simulink model "str_form_iii"  (R2024b)
settings: Solver=FixedStepAuto  StartTime=0.0  StopTime=max_time  FixedStep=Ts  MaxStep=0.02  RelTol=1e-3
undefined symbols (not defined in the file): coa, dVel, goc, K, max_pos, obstacles, offsets, params, pg_period, t_change1, t_change2, Ts, use_col, use_obs, wn_smpl_time
libraries: lib_vehicle_dyn x7
settings Model: Creator=simon  LastModifiedBy=simon
settings RTWCC: GPUComputeCapability=3.5

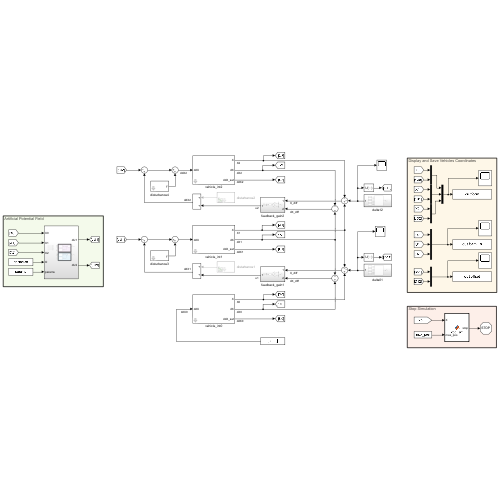
[thumbnail: Simulink's stored preview of the top-level diagram]
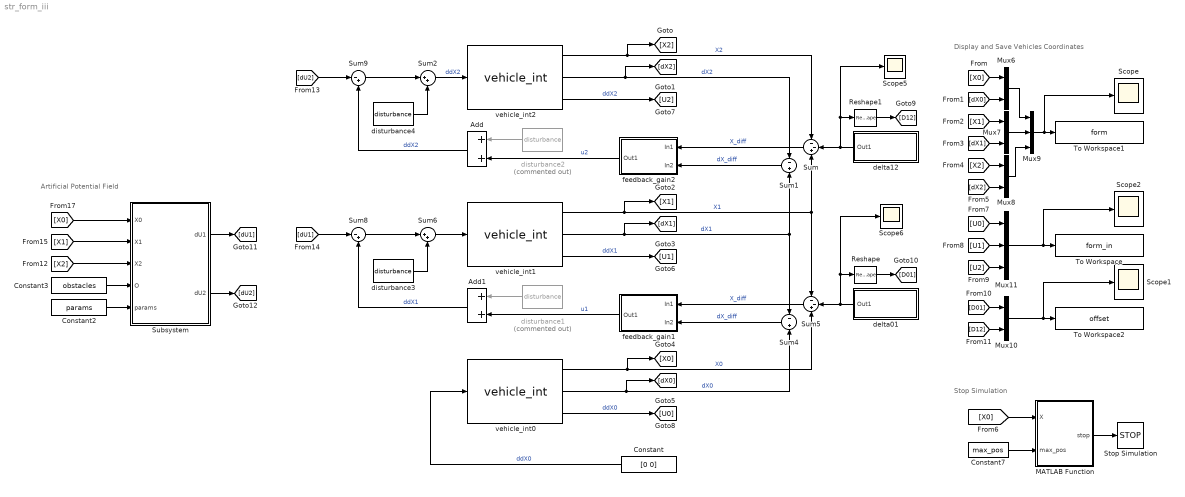
== system str_form_iii ==
  note: Artificial Potential Field
  note: Stop Simulation
  note: Display and Save Vehicles Coordinates
  Add : Sum
  Add1 : Sum
  Constant : Constant  Value=[0 0]
  Constant2 : Constant  Value=params
  Constant3 : Constant  Value=obstacles
  Constant7 : Constant  Value=max_pos
  MATLAB Function : MATLAB Function  TreatAsAtomicUnit=on
  Mux{6..8,10} (4 alike) : Mux  Inputs=2
  Mux11 : Mux  Inputs=3
  Mux9 : Mux  Inputs=3
  Reshape : Reshape
  Reshape1 : Reshape
  Scope{,1..2,5..6} (5 alike) : Scope
  Stop Simulation : Stop
  Subsystem : Subsystem
  Sum : Sum  Inputs=--+
  Sum1 : Sum  Inputs=-+
  Sum2 : Sum  Inputs=|++
  Sum4 : Sum  Inputs=-+
  Sum5 : Sum  Inputs=--+
  Sum6 : Sum  Inputs=|++
  Sum8 : Sum  Inputs=|-+
  Sum9 : Sum  Inputs=|-+
  To Workspace : ToWorkspace  VariableName=form_in  SaveFormat=Structure  SampleTime=Ts
  To Workspace1 : ToWorkspace  VariableName=form  SaveFormat=Structure  SampleTime=Ts
  To Workspace2 : ToWorkspace  VariableName=offset  SaveFormat=Structure  SampleTime=Ts
  delta01 : Subsystem
  delta12 : Subsystem
  disturbance1 : lib_vehicle_dyn/disturbance  Commented=on  wn_amp=wn_amp  wn_smpl_time=wn_smpl_time  wn_gain=wn_gain  pg_amp=pg_amp  pg_period=pg_period  pg_pw=pg_pw  pg_gain=pg_gain
  disturbance2 : lib_vehicle_dyn/disturbance  Commented=on  wn_amp=wn_amp  wn_smpl_time=1/2*wn_smpl_time  wn_gain=wn_gain  pg_amp=pg_amp  pg_period=1/2*pg_period  pg_pw=pg_pw  pg_gain=pg_gain
  disturbance3 : lib_vehicle_dyn/disturbance  wn_amp=wn_amp  wn_smpl_time=wn_smpl_time  wn_gain=wn_gain  pg_amp=pg_amp  pg_period=pg_period  pg_pw=pg_pw  pg_gain=pg_gain
  disturbance4 : lib_vehicle_dyn/disturbance  wn_amp=wn_amp  wn_smpl_time=wn_smpl_time  wn_gain=wn_gain  pg_amp=pg_amp  pg_period=pg_period  pg_pw=pg_pw  pg_gain=pg_gain
  feedback_gain1 : Subsystem
  feedback_gain2 : Subsystem
  vehicle_int0 : lib_vehicle_dyn/vehicle_int  x0=x00  y0=y00  dx0=dx00  dy0=dy00  u_sat=u_sat
  vehicle_int1 : lib_vehicle_dyn/vehicle_int  x0=x10  y0=y10  dx0=dx10  dy0=dy10  u_sat=u_sat
  vehicle_int2 : lib_vehicle_dyn/vehicle_int  x0=x20  y0=y20  dx0=dx20  dy0=dy20  u_sat=u_sat
  wires:
  vehicle_int2/2 -> Sum1/1, [dX2]  "dX2"
  Sum5/1 -> feedback_gain1/1(In1)  "X_diff"
  vehicle_int0/2 -> Sum4/2, [dX0]  "dX0"
  vehicle_int0/1 -> Sum5/3, [X0]  "X0"
  Mux6/1 -> Mux9/1
  [dX2] -> Mux8/2
  Sum1/1 -> feedback_gain2/2(In2)  "dX_diff"
  Sum4/1 -> feedback_gain1/2(In2)  "dX_diff"
  [dX1] -> Mux7/2
  [X1] -> Mux7/1
  feedback_gain1/1(Out1) -> Add1/2  "u1"
  feedback_gain2/1(Out1) -> Add/2  "u2"
  Mux8/1 -> Mux9/3
  [X0] -> Mux6/1
  [X2] -> Mux8/1
  Sum/1 -> feedback_gain2/1(In1)  "X_diff"
  MATLAB Function/1(stop) -> Stop Simulation/1
  [dX0] -> Mux6/2
  [X0] -> MATLAB Function/1(X)
  Constant7/1 -> MATLAB Function/2(max_pos)
  delta12/1(Out1) -> Scope5/1, Reshape1/1, Sum/2
  [U2] -> Mux11/3
  [U0] -> Mux11/1
  [U1] -> Mux11/2
  Mux7/1 -> Mux9/2
  Mux9/1 -> Scope/1, To Workspace1/1
  [D01] -> Mux10/1
  [D12] -> Mux10/2
  Mux10/1 -> Scope1/1, To Workspace2/1
  Mux11/1 -> Scope2/1, To Workspace/1
  Reshape1/1 -> [D12]
  Reshape/1 -> [D01]
  Add/1 -> Sum9/2  "ddX2"
  Add1/1 -> Sum8/2  "ddX1"
  Constant/1 -> vehicle_int0/1  "ddX0"
  vehicle_int2/3 -> [U2]  "ddX2"
  vehicle_int1/3 -> [U1]  "ddX1"
  vehicle_int0/3 -> [U0]  "ddX0"
  vehicle_int1/2 -> Sum4/1, Sum1/2, [dX1]  "dX1"
  Constant2/1 -> Subsystem/5(params)
  [dU1] -> Sum8/1
  Subsystem/2(dU2) -> [dU2]
  Constant3/1 -> Subsystem/4(O)
  [X2] -> Subsystem/3(X2)
  [X0] -> Subsystem/1(X0)
  [X1] -> Subsystem/2(X1)
  Subsystem/1(dU1) -> [dU1]
  vehicle_int2/1 -> [X2], Sum/1  "X2"
  vehicle_int1/1 -> [X1], Sum/3, Sum5/1  "X1"
  Sum6/1 -> vehicle_int1/1
  delta01/1(Out1) -> Scope6/1, Reshape/1, Sum5/2
  [dU2] -> Sum9/1
  disturbance2/1 -> Add/1
  disturbance1/1 -> Add1/1
  Sum2/1 -> vehicle_int2/1  "ddX2"
  Sum9/1 -> Sum2/1
  disturbance4/1 -> Sum2/2
  disturbance3/1 -> Sum6/2
  Sum8/1 -> Sum6/1

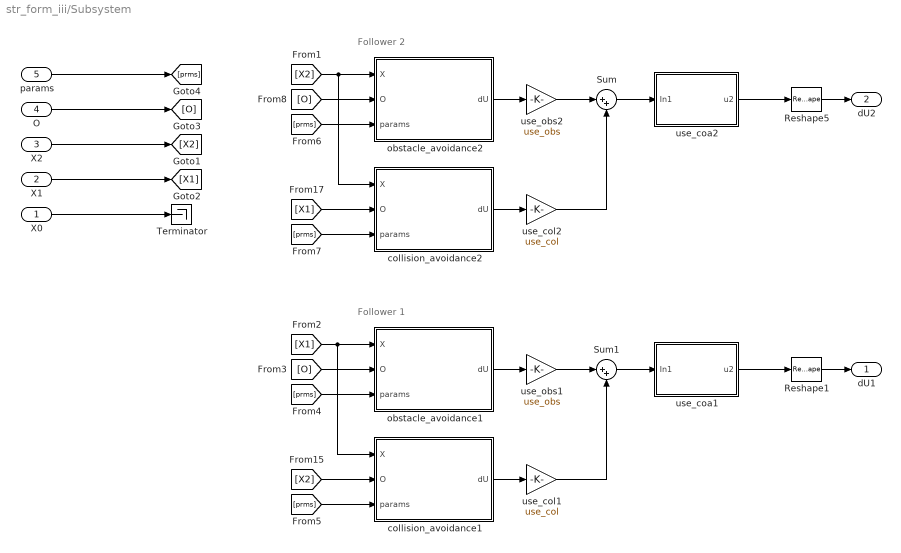
== system str_form_iii/Subsystem ==
  note: Follower 2
  note: Follower 1
  X0 : Inport
  X1 : Inport  Port=2
  X2 : Inport  Port=3
  O : Inport  Port=4
  params : Inport  Port=5
  Reshape1 : Reshape
  Reshape5 : Reshape
  Sum : Sum  Inputs=|++
  Sum1 : Sum  Inputs=|++
  Terminator : Terminator
  collision_avoidance1 : MATLAB Function  TreatAsAtomicUnit=on
  collision_avoidance2 : MATLAB Function  TreatAsAtomicUnit=on
  obstacle_avoidance1 : MATLAB Function  TreatAsAtomicUnit=on
  obstacle_avoidance2 : MATLAB Function  TreatAsAtomicUnit=on
  use_coa1 : Subsystem
  use_coa2 : Subsystem
  use_col1 : Gain  Gain=use_col
  use_col2 : Gain  Gain=use_col
  use_obs1 : Gain  Gain=use_obs
  use_obs2 : Gain  Gain=use_obs
  dU1 : Outport
  dU2 : Outport  Port=2
  wires:
  obstacle_avoidance2/1(dU) -> use_obs2/1
  Sum/1 -> use_coa2/1(In1)
  use_coa2/1(u2) -> Reshape5/1
  use_coa1/1(u2) -> Reshape1/1
  Sum1/1 -> use_coa1/1(In1)
  obstacle_avoidance1/1(dU) -> use_obs1/1
  X2/1 -> [X2]
  X1/1 -> [X1]
  params/1 -> [prms]
  collision_avoidance1/1(dU) -> use_col1/1
  collision_avoidance2/1(dU) -> use_col2/1
  X0/1 -> Terminator/1
  [X1] -> obstacle_avoidance1/1(X), collision_avoidance1/1(X)
  [prms] -> obstacle_avoidance1/3(params)
  [prms] -> collision_avoidance1/3(params)
  [prms] -> obstacle_avoidance2/3(params)
  [prms] -> collision_avoidance2/3(params)
  [O] -> obstacle_avoidance1/2(O)
  [O] -> obstacle_avoidance2/2(O)
  O/1 -> [O]
  [X2] -> collision_avoidance2/1(X), obstacle_avoidance2/1(X)
  use_obs2/1 -> Sum/1
  use_obs1/1 -> Sum1/1
  [X2] -> collision_avoidance1/2(O)
  [X1] -> collision_avoidance2/2(O)
  use_col2/1 -> Sum/2
  use_col1/1 -> Sum1/2
  Reshape5/1 -> dU2/1
  Reshape1/1 -> dU1/1

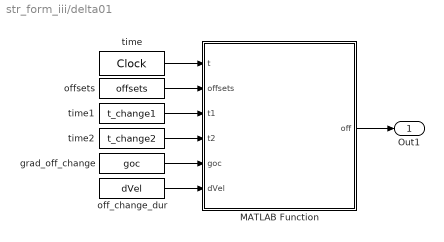
== system str_form_iii/delta01 ==
  MATLAB Function : MATLAB Function  TreatAsAtomicUnit=on
  grad_off_change : Constant  Value=goc
  off_change_dur : Constant  Value=dVel
  offsets : Constant  Value=offsets
  time : DigitalClock  SampleTime=Ts
  time1 : Constant  Value=t_change1
  time2 : Constant  Value=t_change2
  Out1 : Outport  PortDimensions=[2,1]
  wires:
  MATLAB Function/1(off) -> Out1/1
  time2/1 -> MATLAB Function/4(t2)
  offsets/1 -> MATLAB Function/2(offsets)
  time1/1 -> MATLAB Function/3(t1)
  grad_off_change/1 -> MATLAB Function/5(goc)
  time/1 -> MATLAB Function/1(t)
  off_change_dur/1 -> MATLAB Function/6(dVel)

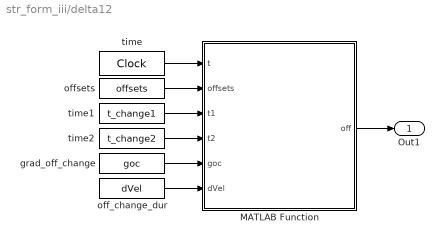
== system str_form_iii/delta12 ==
  MATLAB Function : MATLAB Function  TreatAsAtomicUnit=on
  grad_off_change : Constant  Value=goc
  off_change_dur : Constant  Value=dVel
  offsets : Constant  Value=offsets
  time : DigitalClock  SampleTime=Ts
  time1 : Constant  Value=t_change1
  time2 : Constant  Value=t_change2
  Out1 : Outport  PortDimensions=[2,1]
  wires:
  MATLAB Function/1(off) -> Out1/1
  time/1 -> MATLAB Function/1(t)
  off_change_dur/1 -> MATLAB Function/6(dVel)
  time2/1 -> MATLAB Function/4(t2)
  grad_off_change/1 -> MATLAB Function/5(goc)
  time1/1 -> MATLAB Function/3(t1)
  offsets/1 -> MATLAB Function/2(offsets)

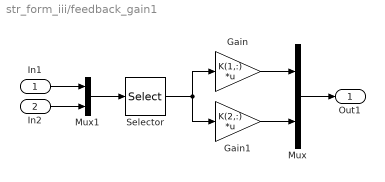
== system str_form_iii/feedback_gain1 ==
  In1 : Inport
  In2 : Inport  Port=2
  Gain : Gain  Gain=K(1,:)  Multiplication=Matrix(K*u)
  Gain1 : Gain  Gain=K(2,:)  Multiplication=Matrix(K*u)
  Mux : Mux  Inputs=2
  Mux1 : Mux  Inputs=2
  Selector : Selector  InputPortWidth=4  IndexOptions=Index vector (dialog)  Indices=[1 3 2 4]  OutputSizes=1
  Out1 : Outport
  wires:
  Mux/1 -> Out1/1
  In1/1 -> Mux1/1
  In2/1 -> Mux1/2
  Mux1/1 -> Selector/1
  Gain/1 -> Mux/1
  Gain1/1 -> Mux/2
  Selector/1 -> Gain/1, Gain1/1

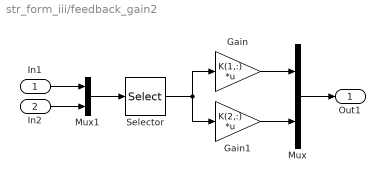
== system str_form_iii/feedback_gain2 ==
  In1 : Inport
  In2 : Inport  Port=2
  Gain : Gain  Gain=K(1,:)  Multiplication=Matrix(K*u)
  Gain1 : Gain  Gain=K(2,:)  Multiplication=Matrix(K*u)
  Mux : Mux  Inputs=2
  Mux1 : Mux  Inputs=2
  Selector : Selector  InputPortWidth=4  IndexOptions=Index vector (dialog)  Indices=[1 3 2 4]  OutputSizes=1
  Out1 : Outport
  wires:
  Mux/1 -> Out1/1
  In1/1 -> Mux1/1
  In2/1 -> Mux1/2
  Mux1/1 -> Selector/1
  Gain/1 -> Mux/1
  Gain1/1 -> Mux/2
  Selector/1 -> Gain/1, Gain1/1

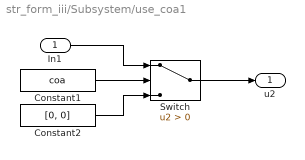
== system str_form_iii/Subsystem/use_coa1 ==
  In1 : Inport
  Constant1 : Constant  Value=coa
  Constant2 : Constant  Value=[0, 0]
  Switch : Switch  Criteria=u2 > Threshold  SaturateOnIntegerOverflow=off  InputSameDT=off
  u2 : Outport
  wires:
  In1/1 -> Switch/1
  Constant1/1 -> Switch/2
  Switch/1 -> u2/1
  Constant2/1 -> Switch/3

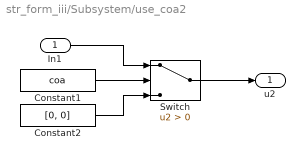
== system str_form_iii/Subsystem/use_coa2 ==
  In1 : Inport
  Constant1 : Constant  Value=coa
  Constant2 : Constant  Value=[0, 0]
  Switch : Switch  Criteria=u2 > Threshold  SaturateOnIntegerOverflow=off  InputSameDT=off
  u2 : Outport
  wires:
  In1/1 -> Switch/1
  Constant1/1 -> Switch/2
  Constant2/1 -> Switch/3
  Switch/1 -> u2/1

== matlab function str_form_iii/delta01/MATLAB Function ==
  data: t input; offsets input size=[2,6]; t1 input; t2 input; goc input; dVel input; off output
function off = variable_offset(t, offsets, t1, t2, goc, dVel)
    % get all offsets between first and second agent
    init_delta = offsets(:,1);
    l2h_delta  = offsets(:,3);
    h2l_delta  = offsets(:,5);

    goc_t1 = norm(init_delta - l2h_delta)/dVel;
    goc_t2 = norm(l2h_delta - h2l_delta)/dVel;

    % time-varying offset with smooth transition using convex combination
    if goc
        if t < t1
            off = init_delta; 
        elseif t >= t1 && t < (t1 + goc_t1)
            i = (t - t1)/goc_t1; 
            off = i.*l2h_delta + (1 - i).*init_delta;
        elseif t >= (t1 + goc_t1) && t < t2
            off = l2h_delta; 
        elseif t >= t2 && t < (t2 + goc_t2)
            i = (t - t2)/goc_t2;
            off = i.*h2l_delta + (1 - i).*l2h_delta;
        else
            off = h2l_delta;
        end
    % time-varying step offset
    else
        off = init_delta;
        if t >= t1
            off = l2h_delta;
        end
        if t >= t2
            off = h2l_delta;
        end
    end
end

== matlab function str_form_iii/MATLAB Function ==
  data: X input; stop output; max_pos input
function stop = stop_sim(X, max_pos)
    stop = 0;
    eps = 1;

    x_max = max_pos(1);
    y_max = max_pos(2);
    
    if sqrt((X(1) - x_max)^2 + (X(2) - y_max)^2) < eps
        stop = 1;
    end
end

== matlab function str_form_iii/delta12/MATLAB Function ==
  data: t input; offsets input size=[2,6]; t1 input; t2 input; goc input; dVel input; off output
function off = variable_offset(t, offsets, t1, t2, goc, dVel)
    % get all offsets between first and second agent
    delta_init = offsets(:,2);
    delta_1  = offsets(:,4);
    delta_2  = offsets(:,6);

    goc_t1 = norm(delta_init - delta_1)/dVel;
    goc_t2 = norm(delta_1 - delta_2)/dVel;

    % time-varying offset with smooth transition using convex combination
    if goc
        if t < t1
            off = delta_init; 
        elseif t >= t1 && t < (t1 + goc_t1)
            i = (t - t1)/goc_t1; 
            off = i.*delta_1 + (1 - i).*delta_init;
        elseif t >= (t1 + goc_t1) && t < t2
            off = delta_1; 
        elseif t >= t2 && t < (t2 + goc_t2)
            i = (t - t2)/goc_t2;
            off = i.*delta_2 + (1 - i).*delta_1;
        else
            off = delta_2;
        end
    % time-varying step offset
    else
        off = delta_init;
        if t >= t1
            off = delta_1;
        end
        if t >= t2
            off = delta_2;
        end
    end
end

== matlab function str_form_iii/Subsystem/collision_avoidance1 ==
  data: X input; dU output; O input; params input
function dU = col_avoid(X, O, params)
    % follower 1 -> avoid follower 2

    eta = params(1);
    rho = params(2);
    q = params(3);
    R = params(4);

    dU = zeros(2,1);

    dx = X(1) - O(1);
    dy = X(2) - O(2);
    r = hypot(dx, dy);
    r_safe = max(r, 1e-9);

    exp_arg = -((r - R)/rho)^q;
    % limit exponential function
    exp_arg = max(min(exp_arg, 60), -60);
    dU_dr = -q*eta*((r - R)^(q - 1))/(rho^q)*exp(exp_arg);

    dU(1) = dU_dr*dx/r_safe;
    dU(2) = dU_dr*dy/r_safe;
end

== matlab function str_form_iii/Subsystem/obstacle_avoidance2 ==
  data: X input; dU output; O input; params input
function dU = obs_avoid(X, O, params)

    eta = params(1);
    rho = params(2);
    q = params(3);
    
    dU = zeros(2,1);

    for i = 1:size(O,2)
        sigma = O(1:2,i);
        R = O(3,i);

        dx = X(1) - sigma(1);
        dy = X(2) - sigma(2);
        r = hypot(dx, dy);
        r_safe = max(r, 1e-9);

        exp_arg = -((r - R)/rho)^q;
        % limit exponential function
        exp_arg = max(min(exp_arg, 60), -60);
        dU_dr = -q*eta*((r - R)^(q - 1))/(rho^q)*exp(exp_arg);
    
        dU(1) = dU(1) + dU_dr*dx/r_safe;
        dU(2) = dU(2) + dU_dr*dy/r_safe;

        % s_raw = r - R;  % signed distance from the boundary
        % s = abs(s_raw); % nonnegative distance to boundary
        % sgn = 1.0; if s_raw < 0, sgn = -1.0; end
        % 
        % % dU/ds: radial derivative wrt s = |r-R|
        % dU_ds = -q*eta*s^(q-1)/rho^q*exp(-(s/rho)^q);
        % dU_dr = sgn*dU_ds;
    end
end

== matlab function str_form_iii/Subsystem/collision_avoidance2 ==
  data: X input; dU output; O input; params input
function dU = col_avoid(X, O, params)
    % follower 2 -> avoid follower 1

    eta = params(1);
    rho = params(2);
    q = params(3);
    R = params(4);

    dU = zeros(2,1);

    dx = X(1) - O(1);
    dy = X(2) - O(2);
    r = hypot(dx, dy);
    r_safe = max(r, 1e-9);

    exp_arg = -((r - R)/rho)^q;
    % limit exponential function
    exp_arg = max(min(exp_arg, 60), -60);
    dU_dr = -q*eta*((r - R)^(q - 1))/(rho^q)*exp(exp_arg);

    dU(1) = dU_dr*dx/r_safe;
    dU(2) = dU_dr*dy/r_safe;
end

== matlab function str_form_iii/Subsystem/obstacle_avoidance1 ==
  data: X input; dU output; O input; params input
function dU = obs_avoid(X, O, params)

    eta = params(1);
    rho = params(2);
    q = params(3);

    dU = zeros(2,1);

    for i = 1:size(O,2)
        sigma = O(1:2,i);
        R = O(3,i);

        dx = X(1) - sigma(1);
        dy = X(2) - sigma(2);
        r = hypot(dx, dy);
        r_safe = max(r, 1e-9);

        exp_arg = -((r - R)/rho)^q;
        % limit exponential function
        exp_arg = max(min(exp_arg, 60), -60);
        dU_dr = -q*eta*((r - R)^(q - 1))/(rho^q)*exp(exp_arg);
    
        dU(1) = dU(1) + dU_dr*dx/r_safe;
        dU(2) = dU(2) + dU_dr*dy/r_safe;

        % s_raw = r - R;  % signed distance from the boundary
        % s = abs(s_raw); % nonnegative distance to boundary
        % sgn = 1.0; if s_raw < 0, sgn = -1.0; end
        % 
        % % dU/ds: radial derivative wrt s = |r-R|
        % dU_ds = -q*eta*s^(q-1)/rho^q*exp(-(s/rho)^q);
        % dU_dr = sgn*dU_ds;
    end
end
